simulink model "Convertidor_planitud_sim"  (R2025b)
settings: Solver=ode45  StartTime=0.0  StopTime=tf  MaxStep=1e-5  RelTol=1e-8  AbsTol=1e-10
undefined symbols (not defined in the file): a_g, k_lc, par, T, t0, x0, y_p, y_q
settings Model: Creator=User  LastModifiedBy=User

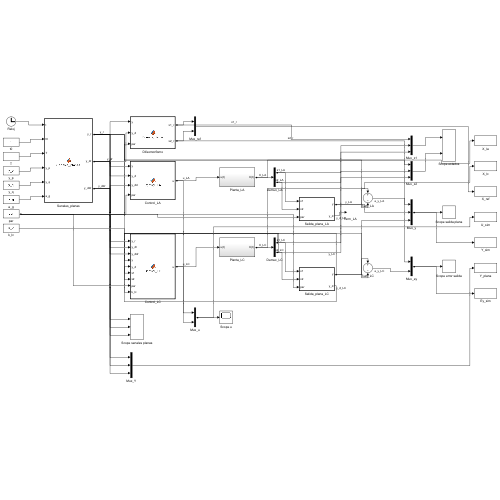
[thumbnail: Simulink's stored preview of the top-level diagram]
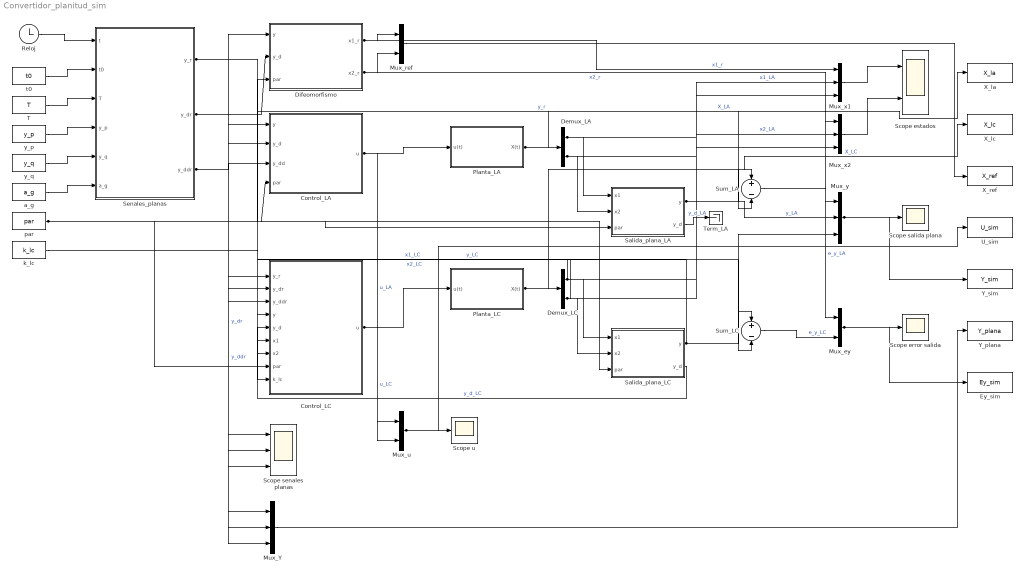
== system Convertidor_planitud_sim ==
  Control_LA : MATLAB Function  TreatAsAtomicUnit=on
  Control_LC : MATLAB Function  TreatAsAtomicUnit=on
  Demux_LA : Demux  Outputs=2
  Demux_LC : Demux  Outputs=2
  Difeomorfismo : MATLAB Function  TreatAsAtomicUnit=on
  Ey_sim : ToWorkspace  VariableName=Ey_sim  SaveFormat=Timeseries  SampleTime=-1
  Mux_Y : Mux  Inputs=3
  Mux_ey : Mux  Inputs=2
  Mux_ref : Mux  Inputs=2
  Mux_u : Mux  Inputs=2
  Mux_x1 : Mux  Inputs=3
  Mux_x2 : Mux  Inputs=3
  Mux_y : Mux  Inputs=3
  Planta_LA : Subsystem
  Planta_LC : Subsystem
  Reloj : Clock
  Salida_plana_LA : MATLAB Function  TreatAsAtomicUnit=on
  Salida_plana_LC : MATLAB Function  TreatAsAtomicUnit=on
  Scope error salida : Scope
  Scope estados : Scope  NumInputPorts=2
  Scope salida plana : Scope
  Scope senales planas : Scope  NumInputPorts=3
  Scope u : Scope
  Senales_planas : MATLAB Function  TreatAsAtomicUnit=on
  Sum_LA : Sum  Inputs=+-
  Sum_LC : Sum  Inputs=+-
  T : Constant  Value=T
  Term_LA : Terminator
  U_sim : ToWorkspace  VariableName=U_sim  SaveFormat=Timeseries  SampleTime=-1
  X_la : ToWorkspace  VariableName=X_la  SaveFormat=Timeseries  SampleTime=-1
  X_lc : ToWorkspace  VariableName=X_lc  SaveFormat=Timeseries  SampleTime=-1
  X_ref : ToWorkspace  VariableName=X_ref  SaveFormat=Timeseries  SampleTime=-1
  Y_plana : ToWorkspace  VariableName=Y_plana  SaveFormat=Timeseries  SampleTime=-1
  Y_sim : ToWorkspace  VariableName=Y_sim  SaveFormat=Timeseries  SampleTime=-1
  a_g : Constant  Value=a_g
  k_lc : Constant  Value=k_lc
  par : Constant  Value=par
  t0 : Constant  Value=t0
  y_p : Constant  Value=y_p
  y_q : Constant  Value=y_q
  wires:
  Reloj/1 -> Senales_planas/1(t)
  t0/1 -> Senales_planas/2(t0)
  T/1 -> Senales_planas/3(T)
  y_p/1 -> Senales_planas/4(y_p)
  y_q/1 -> Senales_planas/5(y_q)
  a_g/1 -> Senales_planas/6(a_g)
  Senales_planas/1(y_r) -> Difeomorfismo/1(y), Control_LA/1(y), Control_LC/1(y_r), Sum_LA/2, Sum_LC/2, Scope senales planas/1, Mux_y/1, Mux_Y/1  "y_r"
  Senales_planas/2(y_dr) -> Difeomorfismo/2(y_d), Control_LA/2(y_d), Control_LC/2(y_dr), Scope senales planas/2, Mux_Y/2  "y_dr"
  Senales_planas/3(y_ddr) -> Control_LA/3(y_dd), Control_LC/3(y_ddr), Scope senales planas/3, Mux_Y/3  "y_ddr"
  par/1 -> Difeomorfismo/3(par), Control_LA/4(par), Salida_plana_LA/3(par), Salida_plana_LC/3(par), Control_LC/8(par)
  Control_LA/1(u) -> Planta_LA/1(u(t)), Mux_u/1  "u_LA"
  Planta_LA/1(X(t)) -> Demux_LA/1, X_la/1  "X_LA"
  Planta_LC/1(X(t)) -> Demux_LC/1, X_lc/1  "X_LC"
  Demux_LA/1 -> Salida_plana_LA/1(x1), Mux_x1/2  "x1_LA"
  Demux_LC/1 -> Salida_plana_LC/1(x1), Control_LC/6(x1), Mux_x1/3  "x1_LC"
  Demux_LA/2 -> Salida_plana_LA/2(x2), Mux_x2/2  "x2_LA"
  Demux_LC/2 -> Salida_plana_LC/2(x2), Control_LC/7(x2), Mux_x2/3  "x2_LC"
  Salida_plana_LC/1(y) -> Control_LC/4(y), Sum_LC/1, Mux_y/3  "y_LC"
  Salida_plana_LC/2(y_d) -> Control_LC/5(y_d)  "y_d_LC"
  k_lc/1 -> Control_LC/9(k_lc)
  Control_LC/1(u) -> Planta_LC/1(u(t)), Mux_u/2  "u_LC"
  Salida_plana_LA/2(y_d) -> Term_LA/1  "y_d_LA"
  Salida_plana_LA/1(y) -> Sum_LA/1, Mux_y/2  "y_LA"
  Mux_u/1 -> Scope u/1, U_sim/1
  Difeomorfismo/1(x1_r) -> Mux_x1/1, Mux_ref/1  "x1_r"
  Mux_x1/1 -> Scope estados/1
  Difeomorfismo/2(x2_r) -> Mux_x2/1, Mux_ref/2  "x2_r"
  Mux_x2/1 -> Scope estados/2
  Mux_y/1 -> Scope salida plana/1, Y_sim/1
  Sum_LA/1 -> Mux_ey/1  "e_y_LA"
  Sum_LC/1 -> Mux_ey/2  "e_y_LC"
  Mux_ey/1 -> Scope error salida/1, Ey_sim/1
  Mux_ref/1 -> X_ref/1
  Mux_Y/1 -> Y_plana/1

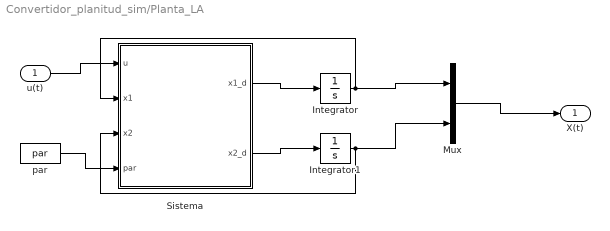
== system Convertidor_planitud_sim/Planta_LA ==
  u(t) : Inport
  Integrator : Integrator  InitialCondition=x0(1)
  Integrator1 : Integrator  InitialCondition=x0(2)
  Mux : Mux  Inputs=2
  Sistema : MATLAB Function  TreatAsAtomicUnit=on
  par : Constant  Value=par
  X(t) : Outport
  wires:
  u(t)/1 -> Sistema/1(u)
  par/1 -> Sistema/4(par)
  Sistema/1(x1_d) -> Integrator/1
  Integrator/1 -> Sistema/2(x1), Mux/1
  Sistema/2(x2_d) -> Integrator1/1
  Integrator1/1 -> Sistema/3(x2), Mux/2
  Mux/1 -> X(t)/1

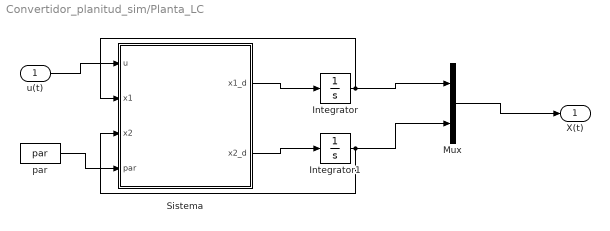
== system Convertidor_planitud_sim/Planta_LC ==
  u(t) : Inport
  Integrator : Integrator  InitialCondition=x0(1)
  Integrator1 : Integrator  InitialCondition=x0(2)
  Mux : Mux  Inputs=2
  Sistema : MATLAB Function  TreatAsAtomicUnit=on
  par : Constant  Value=par
  X(t) : Outport
  wires:
  u(t)/1 -> Sistema/1(u)
  par/1 -> Sistema/4(par)
  Sistema/1(x1_d) -> Integrator/1
  Integrator/1 -> Sistema/2(x1), Mux/1
  Sistema/2(x2_d) -> Integrator1/1
  Integrator1/1 -> Sistema/3(x2), Mux/2
  Mux/1 -> X(t)/1

== matlab function Convertidor_planitud_sim/Difeomorfismo ==
  data: y input; x1_r output; y_d input; par input; x2_r output
function [x1_r, x2_r] = Difeomorfismo(y, y_d, par)

E = par(1); L = par(2); C = par(3); R = par(4);
x1_r = -E*R*C/(2*L) + sqrt((E*R*C/(2*L))^2 + (2*y + R*C*y_d)/L);
x2_r = sqrt(R*(E*x1_r - y_d));

== matlab function Convertidor_planitud_sim/Senales_planas ==
  data: t input; y_r output; t0 input; T input; y_p input; y_q input; a_g input; y_dr output; y_ddr output
function [y_r, y_dr, y_ddr] = Senales_planas(t, t0, T, y_p, y_q, a_g)

tn = min(max((t - t0)/T, 0), 1);

gam  = a_g(1)*tn^3 + a_g(2)*tn^4 + a_g(3)*tn^5;
gam1 = 3*a_g(1)*tn^2 + 4*a_g(2)*tn^3 + 5*a_g(3)*tn^4;
gam2 = 6*a_g(1)*tn + 12*a_g(2)*tn^2 + 20*a_g(3)*tn^3;

Dy    = y_q - y_p;
y_r   = y_p + Dy*gam;
y_dr  = Dy*gam1/T;
y_ddr = Dy*gam2/T^2;

== matlab function Convertidor_planitud_sim/Control_LA ==
  data: y input; u output; y_d input; y_dd input; par input
function u = Control_LA(y, y_d, y_dd, par)

E = par(1); L = par(2); C = par(3); R = par(4);
x1 = -E*R*C/(2*L) + sqrt((E*R*C/(2*L))^2 + (2*y + R*C*y_d)/L);
x2 = sqrt(R*(E*x1 - y_d));
Lf2   = E^2/L + 2*x2^2/(C*R^2);
LgLf1 = -x2*(C*E*R + 2*L*x1)/(C*L*R);
u = (y_dd - Lf2)/LgLf1;

== matlab function Convertidor_planitud_sim/Planta_LA/Sistema ==
  data: u input; x1_d output; x1 input; x2 input; par input; x2_d output
function [x1_d, x2_d] = Sistema(u, x1, x2, par)

E = par(1); L = par(2); C = par(3); R = par(4);
x1_d = -(1/L)*u*x2 + E/L;
x2_d =  (1/C)*u*x1 - (1/(R*C))*x2;

== matlab function Convertidor_planitud_sim/Planta_LC/Sistema ==
  data: u input; x1_d output; x1 input; x2 input; par input; x2_d output
function [x1_d, x2_d] = Sistema(u, x1, x2, par)

E = par(1); L = par(2); C = par(3); R = par(4);
x1_d = -(1/L)*u*x2 + E/L;
x2_d =  (1/C)*u*x1 - (1/(R*C))*x2;

== matlab function Convertidor_planitud_sim/Salida_plana_LA ==
  data: x1 input; y output; x2 input; par input; y_d output
function [y, y_d] = Salida_plana(x1, x2, par)

E = par(1); L = par(2); C = par(3); R = par(4);
y   = 1/2*L*x1^2 + 1/2*C*x2^2;
y_d = E*x1 - x2^2/R;

== matlab function Convertidor_planitud_sim/Salida_plana_LC ==
  data: x1 input; y output; x2 input; par input; y_d output
function [y, y_d] = Salida_plana(x1, x2, par)

E = par(1); L = par(2); C = par(3); R = par(4);
y   = 1/2*L*x1^2 + 1/2*C*x2^2;
y_d = E*x1 - x2^2/R;

== matlab function Convertidor_planitud_sim/Control_LC ==
  data: y_r input; u output; y_dr input; y_ddr input; y input; y_d input; x1 input; x2 input; par input; k_lc input
function u = Control_LC(y_r, y_dr, y_ddr, y, y_d, x1, x2, par, k_lc)

E = par(1); L = par(2); C = par(3); R = par(4);
k0 = k_lc(1); k1 = k_lc(2);
v     = y_ddr - k1*(y_d - y_dr) - k0*(y - y_r);
Lf2   = E^2/L + 2*x2^2/(C*R^2);
LgLf1 = -x2*(C*E*R + 2*L*x1)/(C*L*R);
u     = (v - Lf2)/LgLf1;
